simulink model "Project_Controller"  (R2025b)
settings: Solver=FixedStepDiscrete  StartTime=0.0  StopTime=36  FixedStep=1e-4  RelTol=1e-3
model workspace (MATLAB code in the model file):
  | %% Model workspace of Project_Controller.slx (Data source: MATLAB Code)
  | % The whole design chain, so the model runs on its own: physical parameters -> state-space model
  | % -> LQR with integral action -> Kalman filter -> discretization. Needs Control System Toolbox.
  | % Same computation as plant_model.m + controller_design.m (gain set v3a) + controller_params.m.
  | % build_controller_model.m copies this file into the model and checks it against those files.
  | 
  | %% Test case (same controller for both, no retuning)
  | rHigh = 0.015;   % [m] 0.015 (15 -> 5 mm) or 0.020 (20 -> 5 mm)
  | rLow  = 0.005;   % [m]
  | tHold = 12;      % [s] rLow, rHigh, rLow for tHold s each (stop time = 3*tHold = 36 s)
  | 
  | %% Physical parameters (project description, Table 1)
  | R    = 0.55;      % motor resistance [Ohm]
  | L    = 0.8e-3;    % motor inductance [H]
  | ki   = 0.036;     % torque constant [Nm/A]
  | kb   = 0.036;     % back-emf constant [V/(rad/s)]
  | lead = 0.01;      % ball screw lead [m/rev]
  | eta  = 1;         % ball screw efficiency (prescribed; real value < 1, robustness checked)
  | ma   = 0.3;       % actuator moving mass [kg]
  | ml   = 0.51;      % payload mass [kg]
  | 
  | %% Identified parameters (Section 3 of the report)
  | ks   = 131.66;    % spring [N/m], static stretch test
  | bs   = 0.0048;    % damper [Ns/m], free decay, logarithmic decrement
  | kv   = 0.99;      % input gain relative to Table 1, closed-loop frequency response
  | tauM = 0.018;     % actuator time constant [s], frequency response (Table 1 gives 31 ms)
  | tauS = 0.0106;    % sensor lag [s], Balluff -3 dB at 15 Hz
  | 
  | %% State-space model, deviations from the equilibrium point (plant_model.m)
  | % states [i y ydot x xdot xs]: current, actuator pos/vel, payload pos/vel, sensor state
  | N  = 2*pi/lead;             % screw ratio, omega = N*ydot [rad/m]
  | Kf = eta*N*ki;              % actuator force per ampere [N/A]
  | Kb = kb*N;                  % back emf per actuator speed [V/(m/s)]
  | Me = tauM*Kf*Kb/R;          % effective moving mass that gives tauM = Me*R/(Kf*Kb) [kg]
  | A = [ -R/L     0       -Kb/L     0       0        0
  |          0     0         1       0       0        0
  |      Kf/Me -ks/Me    -bs/Me   ks/Me   bs/Me       0
  |          0     0         0       0       1        0
  |          0  ks/ml     bs/ml  -ks/ml  -bs/ml       0
  |          0     0         0   1/tauS      0  -1/tauS ];
  | B = [kv/L; 0; 0; 0; 0; 0];
  | C = [0 0 0 0 0 1];          % only the (lagged) payload position is measured
  | n = size(A, 1);
  | 
  | %% LQR with integral action (L3d, L3g), Bryson's rule q_ii = 1/x_max^2, r = 1/u_max^2
  | % max: i 5 A, y 25 mm (stroke), ydot 0.15 m/s, x 8 mm, xdot 20 mm/s, xs not weighted,
  | % integral 1 mm*s, voltage 5 V
  | Ai = [A zeros(n, 1); -C 0];
  | Bi = [B; 0];
  | Q  = diag(1 ./ [5 0.025 0.15 0.008 0.02 1e3 0.001].^2);
  | Ru = 1/5^2;
  | Kaug = lqr(Ai, Bi, Q, Ru);
  | K  = Kaug(1:n);             % u = -K*xhat + Ke*xN
  | Ke = -Kaug(n + 1);
  | 
  | %% Kalman filter (LQE, L3h): process noise as voltage (3 V) and payload force (1 N push)
  | G   = [B, [0; 0; 0; 0; 1/ml; 0]];
  | sigX = 22e-6;               % measured sensor noise std [m]
  | [~, Lobs] = kalman(ss(A, [B G], C, 0), diag([3^2, 1^2]), sigX^2);
  | 
  | %% Discretization at the Speedgoat rate. Observer inputs [u; x]
  | Ts = 1e-4;                  % [s]
  | obsD = c2d(ss(A - Lobs*C, [B Lobs], eye(n), 0), Ts);
  | Ao = obsD.A;  Bo = obsD.B;
  | 
  | %% Holding voltage (equilibrium input) and voltage limit
  | vMax   = 5;                 % interface limit [V]
  | vBias  = 0.6;               % measured holding voltage [V]
  | uLim   = [-vMax, vMax];     % limit on u + vBias [V]
  | 
  | %% Reference prefilter 1/(tauPre*s + 1)^2, outside the loop
  | tauPre = 0.3;               % [s]
  | preD = ss(c2d(tf(1, [tauPre^2 2*tauPre 1]), Ts));
  | 
  | %% Start-up from the measured rest position x(0) (it changes between sessions, 1.57-1.85 mm)
  | x0map  = [0; 1; 0; 1; 0; 1];                     % xhat0 = x0map*x(0): positions = x(0), rest
  | preMap = (eye(size(preD.A)) - preD.A) \ preD.B;   % prefilter state in steady state at x(0)
  | 
  | %% Chirp excitation (frequency-response identification) and dither: both off
  | aExc = 0;  tExc = 5;  tExcDur = 60;  fExc1 = 0.3;  fExc2 = 20;
  | aDither = 0;  fDither = 100;
undefined symbols (not defined in the file): DiscIntNeverNeededParam, Pull, up
libraries: speedgoatlib_IO183 x3, simulink x1
settings Model: SimulationMode=external  Creator=rafaeltavares  LastModifiedBy=havard
settings SolverCC: ConcurrentTasks=on  AlgebraicLoopSolver=TrustRegion  PositivePriorityOrder=on  InsertRTBMode=Never (minimum delay)
settings DataIOCC: SaveFormat=StructureWithTime  ReturnWorkspaceOutputs=off
settings OptimizationCC: BlockReduction=off  OptimizeBlockIOStorage=off  BufferReuse=off  GlobalBufferReuse=off  ExpressionFolding=off  LocalBlockOutputs=off  OptimizeDataStoreBuffers=off  BusAssignmentInplaceUpdate=off
settings DebuggingCC: TasksWithSamePriorityMsg=none  UnconnectedInputMsg=warning  UnconnectedOutputMsg=warning  UnconnectedLineMsg=warning  UnderSpecifiedDimensionMsg=warning  ArithmeticOperatorsInVariantConditions=warning
settings HardwareCC: ProdBitPerLong=64.0  ProdLongLongMode=on  ProdHWDeviceType=Intel->x86-64 (Linux 64)
settings ModelReferenceCC: EnableRefExpFcnMdlSchedulingChecks=on
settings SFSimCC: CustomCodeUndefinedFunction=UseInterfaceOnly
settings RTWCC: SystemTargetFile=speedgoat.tlc  TemplateMakefile=slrealtime_default_tmf  Toolchain=Simulink Real-Time Toolchain  BuildConfiguration=Faster Runs  CodeExecutionProfiling=on  TargetLang=C++  GPUComputeCapability=3.5  DLArmComputeVersion=19.05  Description=Speedgoat Real-Time Target Machine
settings SimulinkRealTimeTargetCC: SLRTFileLogMaxRuns=1.0  ExtModeMaxTrigDuration=10.0  ExtModeStaticAllocSize=1000000.0  ExtModeTransport=0.0  MultiwordLength=2048.0  DynamicStringBufferSize=256.0  PreserveMATLABNamespacesInGeneratedCode=on  SubcomponentCodeInterfacePackaging=Reusable function  InstructionSetFMA=off  LogToMDFFile=off

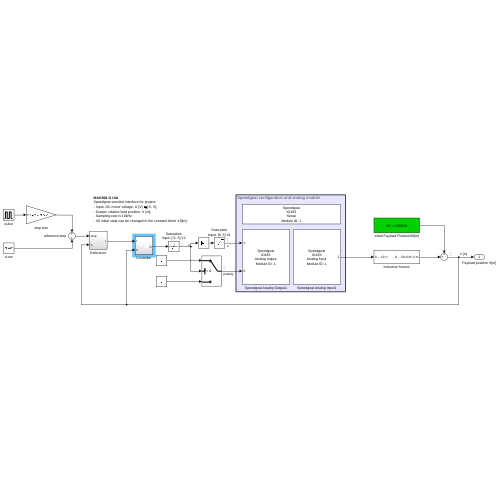
[thumbnail: Simulink's stored preview of the top-level diagram]
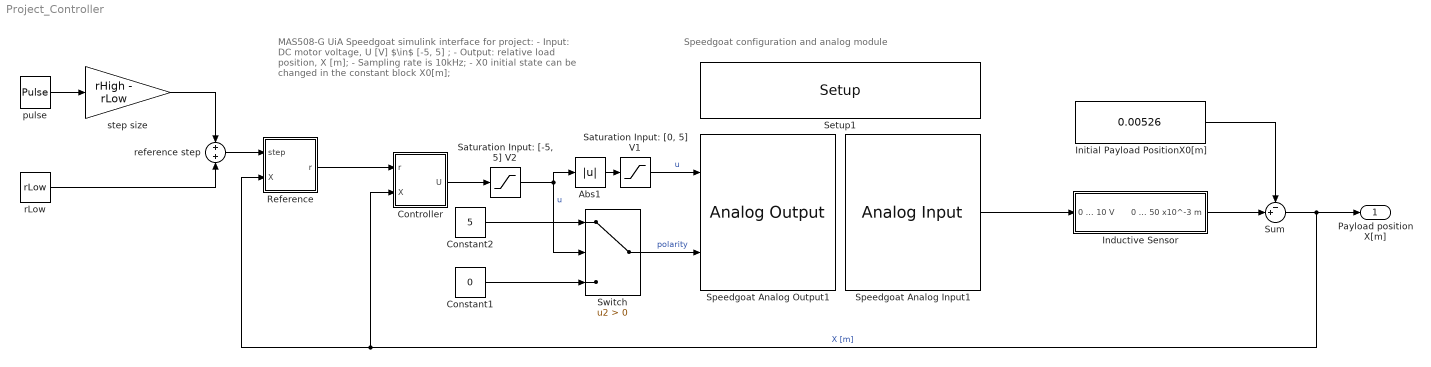
== system Project_Controller ==
  note: MAS508-G UiA
      | Speedgoat simulink interface for project:
      | - Input: DC motor voltage, U [V] $\in$ [-5, 5] ;
      | - Output: relative load position, X [m];
      | - Sampling rate is 10kHz;
      | - X0 initial state can be changed in the constant block X0[m];
  note: Speedgoat configuration and analog module
  Abs1 : Abs  SaturateOnIntegerOverflow=off
  Constant1 : Constant  Value=0
  Constant2 : Constant  Value=5
  Controller : Subsystem
  "Inductive Sensor " : Subsystem
  "Initial Payload PositionX0[m] " : Constant  Value=0.00526
      mask Display:
      | set_param(gcb,'BackgroundColor','green');
      | fprintf('X0 = %s', get_param(gcb,'Value'))
  Reference : Subsystem
  "Saturation Input: [-5, 5] V2" : Saturate  UpperLimit=5  LowerLimit=-5
  "Saturation Input: [0, 5] V1" : Saturate  UpperLimit=5  LowerLimit=0
  Setup1 : speedgoatlib_IO183/Setup  parModuleId=1  parPciSlot=-1  parDaSimult=on  parAdCoupling=Single Ended  parAdRange=0..10V  parAdChannelLow=1  parAdChannelHigh=1  parDaChannels=[1 2]  parDaRange=0..5V  parDaInit=[0 5 0 0]  parDaReset=1  parDoChannels=[1:8]  parDoInit=[0]  parDoReset=[1]  parDiChannels=[9:16]  parIOPullReferenceFront=Pull-up (3.3V)  parIOPullReferenceRear=Pull-up (3.3V)
      settings: SourceProductName=IO183
  Speedgoat Analog Input1 : speedgoatlib_IO183/Analog Input  Priority=0  parModuleId=1  parSampTime=-1  parPciSlot=-1  parAdChannelLow=1  parAdChannelHigh=1
      settings: SourceProductName=IO183
  Speedgoat Analog Output1 : speedgoatlib_IO183/Analog Output  parModuleId=1  parSampTime=-1  parDaSimult=on  parPciSlot=-1  parDaChannels=[1 2]  parDaInit=[0 5 0 0]  parDaReset=[1 1 1 1]
      settings: SourceProductName=IO183
  Sum : Sum  Inputs=-+|
  Switch : Switch  Criteria=u2 > Threshold  SaturateOnIntegerOverflow=off  InputSameDT=off
  pulse : DiscretePulseGenerator  PulseType=Time based  Period=2*tHold  PulseWidth=50  PhaseDelay=tHold
  rLow : Constant  Value=rLow
  reference step : Sum
  step size : Gain  Gain=rHigh - rLow
  Payload position X[m] : Outport
  wires:
  "Inductive Sensor "/1(0 ... 50 x10^-3 m) -> Sum/2
  "Initial Payload PositionX0[m] "/1 -> Sum/1
  "Saturation Input: [0, 5] V1"/1 -> Speedgoat Analog Output1/1  "u"
  Constant2/1 -> Switch/1
  Speedgoat Analog Input1/1 -> "Inductive Sensor "/1(0 ... 10 V)
  Abs1/1 -> "Saturation Input: [0, 5] V1"/1
  Switch/1 -> Speedgoat Analog Output1/2  "polarity"
  Constant1/1 -> Switch/3
  "Saturation Input: [-5, 5] V2"/1 -> Abs1/1, Switch/2  "u"
  Sum/1 -> Reference/2(X), Controller/2(X), Payload position X[m]/1  "X [m]"
  pulse/1 -> step size/1
  step size/1 -> reference step/1
  rLow/1 -> reference step/2
  reference step/1 -> Reference/1(step)
  Reference/1(r) -> Controller/1(r)
  Controller/1(U) -> "Saturation Input: [-5, 5] V2"/1

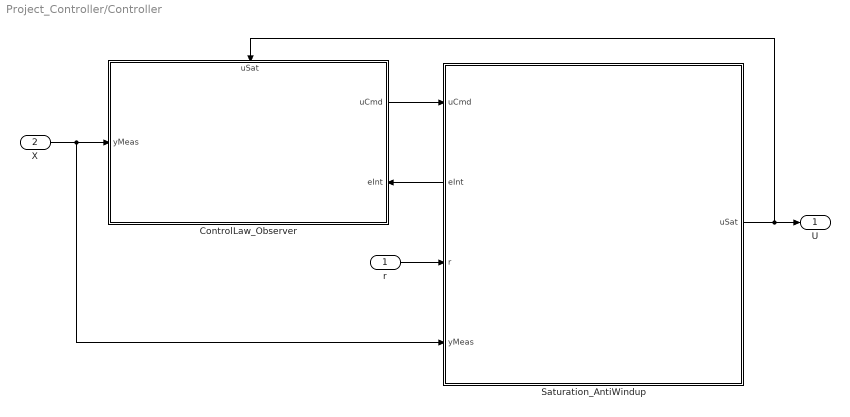
== system Project_Controller/Controller ==
  r : Inport
  X : Inport  Port=2
  ControlLaw_Observer : Subsystem
      settings: PortSchema="{\"entries\":[{\"content\":{\"sides\":[{\"content\":{\"connectorIds\":[\"In1\"]},\"type\":\"ConnectorPlacement.EquallySpacedRectSide\",\"uuid\":\"4ab0fcb8-52c7-4a4e-9377-be86be06758b\"},{\"content\":{\"connectorIds\":[\"Out1\",\"In3\"],\"side\":\"RIGHT\"},\"type\":\"ConnectorPlacement.EquallySpacedRectSide\",\"uuid\":\"0c93ed77-db89-4914-8ed3-cc59a8eb3b85\"},{\"content\":{\"connectorIds\":[\"In2\"],\"side\":\"TOP\"},\"type\":\"ConnectorPlacement.EquallySpacedRectSide\",\"uuid\":\"1c748175-366b-4d57-8d03-3856bbcdfb09\"},{\"content\":{\"side\":\"BOTTOM\"},\"type\":\"ConnectorPlacement.EquallySpacedRectSide\",\"uuid\":\"18ee6780-29bb-4133-baad-5bb614cd70f7\"}]},\"type\":\"ConnectorPlacement.EquallySpacedConnector\",\"uuid\":\"9b829baf-7a37-4ed0-ad0c-dec2a53cf1cf\"}],\"packageUris\":[\"http://schema.mathworks.com/mf0/Connector/R2020b\"],\"version\":\"1.0\"}"
  Saturation_AntiWindup : Subsystem
      settings: PortSchema="{\"entries\":[{\"content\":{\"sides\":[{\"content\":{\"connectorIds\":[\"In1\",\"Out2\",\"In2\",\"In3\"]},\"type\":\"ConnectorPlacement.EquallySpacedRectSide\",\"uuid\":\"fd51be67-1b16-4c80-8941-43d479349b34\"},{\"content\":{\"connectorIds\":[\"Out1\"],\"side\":\"RIGHT\"},\"type\":\"ConnectorPlacement.EquallySpacedRectSide\",\"uuid\":\"50a9a10a-2e08-446e-b14e-5678e3c6d1e3\"},{\"content\":{\"side\":\"TOP\"},\"type\":\"ConnectorPlacement.EquallySpacedRectSide\",\"uuid\":\"8fd36ea3-ab38-479f-a719-6e347c4892f4\"}]},\"type\":\"ConnectorPlacement.EquallySpacedConnector\",\"uuid\":\"95e37cf3-826c-49dc-833f-2565447af58e\"}],\"packageUris\":[\"http://schema.mathworks.com/mf0/Connector/R2020b\"],\"version\":\"1.0\"}"
  U : Outport
  wires:
  r/1 -> Saturation_AntiWindup/2(r)
  X/1 -> ControlLaw_Observer/1(yMeas), Saturation_AntiWindup/3(yMeas)
  ControlLaw_Observer/1(uCmd) -> Saturation_AntiWindup/1(uCmd)
  Saturation_AntiWindup/1(uSat) -> U/1, ControlLaw_Observer/2(uSat)
  Saturation_AntiWindup/2(eInt) -> ControlLaw_Observer/3(eInt)

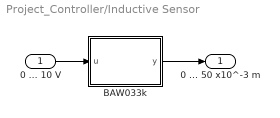
== system Project_Controller/Inductive Sensor  ==
  0 ... 10 V : Inport
  BAW033k : MATLAB Function  TreatAsAtomicUnit=on
  0 ... 50 x10^-3 m : Outport  VectorParamsAs1DForOutWhenUnconnected=off
  wires:
  BAW033k/1(y) -> 0 ... 50 x10^-3 m/1
  0 ... 10 V/1 -> BAW033k/1(u)

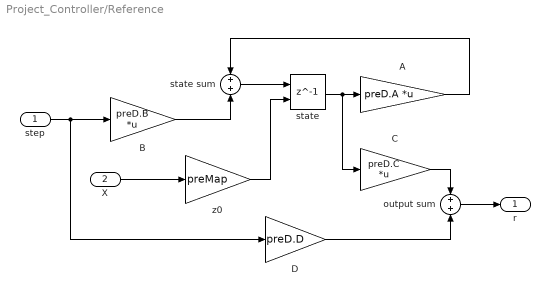
== system Project_Controller/Reference ==
  step : Inport
  X : Inport  Port=2
  A : Gain  Gain=preD.A  Multiplication=Matrix(K*u)
  B : Gain  Gain=preD.B  Multiplication=Matrix(K*u)
  C : Gain  Gain=preD.C  Multiplication=Matrix(K*u)
  D : Gain  Gain=preD.D
  output sum : Sum
  state : Delay  DelayLength=1  InitialConditionSource=Input port  SampleTime=Ts
      settings: InputPortMap=u0,p4
  state sum : Sum
  z0 : Gain  Gain=preMap
  r : Outport
  wires:
  output sum/1 -> r/1
  A/1 -> state sum/1
  state/1 -> C/1, A/1
  z0/1 -> state/2
  X/1 -> z0/1
  C/1 -> output sum/1
  D/1 -> output sum/2
  B/1 -> state sum/2
  state sum/1 -> state/1
  step/1 -> B/1, D/1

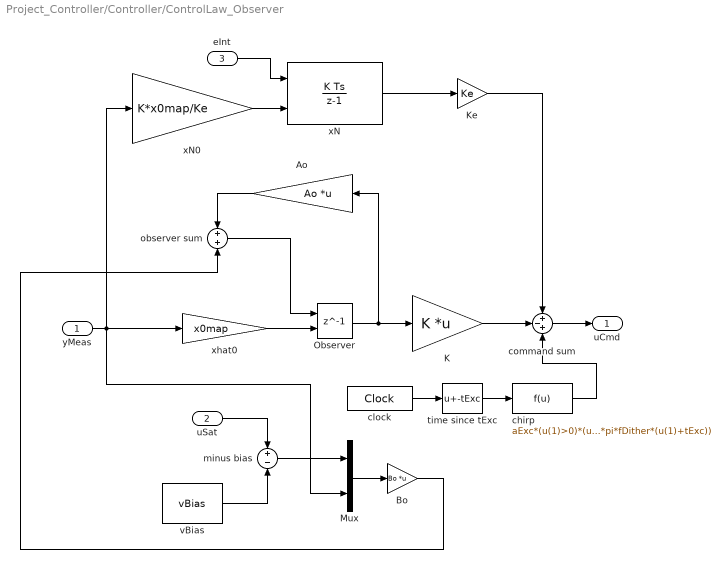
== system Project_Controller/Controller/ControlLaw_Observer ==
  yMeas : Inport
  uSat : Inport  Port=2
  eInt : Inport  Port=3
  Ao : Gain  Gain=Ao  Multiplication=Matrix(K*u)
  Bo : Gain  Gain=Bo  Multiplication=Matrix(K*u)
  K : Gain  Gain=K  Multiplication=Matrix(K*u)
  Ke : Gain  Gain=Ke
  Mux : Mux  Inputs=2
  Observer : Delay  DelayLength=1  InitialConditionSource=Input port  SampleTime=Ts
      settings: InputPortMap=u0,p4
  chirp : Fcn  Expr=aExc*(u(1)>0)*(u(1)<tExcDur)*sin(2*pi*(fExc1*u(1) + (fExc2-fExc1)/(2*tExcDur)*u(1)^2)) + aDither*sin(2*pi*fDither*(u(1)+tExc))
  clock : DigitalClock  SampleTime=Ts
  command sum : Sum  Inputs=+-+
  minus bias : Sum  Inputs=+-
  observer sum : Sum
  time since tExc : Bias  Bias=-tExc  SaturateOnIntegerOverflow=off
  vBias : Constant  Value=vBias
  xN : DiscreteIntegrator  InitialConditionSource=external  SampleTime=Ts  ICPrevOutput=DiscIntNeverNeededParam  ICPrevScaledInput=DiscIntNeverNeededParam
  xN0 : Gain  Gain=K*x0map/Ke
  xhat0 : Gain  Gain=x0map
  uCmd : Outport
  wires:
  Ke/1 -> command sum/1
  eInt/1 -> xN/1
  xhat0/1 -> Observer/2
  yMeas/1 -> Mux/2, xhat0/1, xN0/1
  command sum/1 -> uCmd/1
  Observer/1 -> Ao/1, K/1
  xN0/1 -> xN/2
  Ao/1 -> observer sum/1
  xN/1 -> Ke/1
  K/1 -> command sum/2
  observer sum/1 -> Observer/1
  uSat/1 -> minus bias/1
  vBias/1 -> minus bias/2
  minus bias/1 -> Mux/1
  Mux/1 -> Bo/1
  Bo/1 -> observer sum/2
  time since tExc/1 -> chirp/1
  chirp/1 -> command sum/3
  clock/1 -> time since tExc/1

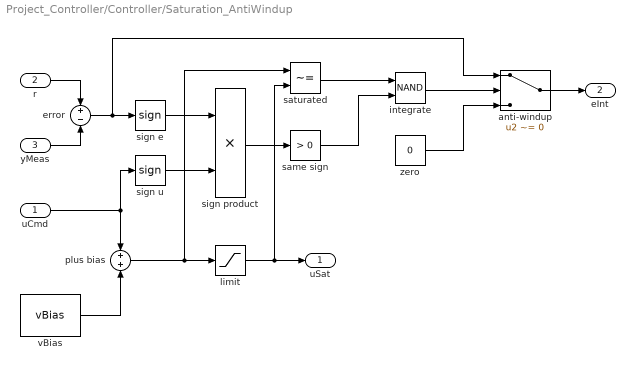
== system Project_Controller/Controller/Saturation_AntiWindup ==
  uCmd : Inport
  r : Inport  Port=2
  yMeas : Inport  Port=3
  anti-windup : Switch  Criteria=u2 ~= 0  SaturateOnIntegerOverflow=off  InputSameDT=off
  error : Sum  Inputs=+-
  integrate : Logic  Operator=NAND  AllPortsSameDT=off  OutDataTypeStr=boolean
  limit : Saturate  UpperLimit=uLim(2)  LowerLimit=uLim(1)
  plus bias : Sum
  same sign : simulink/Logic and Bit Operations/Compare To Constant  relop=>  const=0  OutDataTypeStr=boolean
  saturated : RelationalOperator  Operator=~=  OutDataTypeStr=boolean  RndMeth=Simplest  InputSameDT=off
  sign e : Signum
  sign product : Product
  sign u : Signum
  vBias : Constant  Value=vBias
  zero : Constant  Value=0
  uSat : Outport
  eInt : Outport  Port=2
  wires:
  same sign/1 -> integrate/2
  sign u/1 -> sign product/2
  integrate/1 -> anti-windup/2
  yMeas/1 -> error/2
  saturated/1 -> integrate/1
  anti-windup/1 -> eInt/1
  uCmd/1 -> plus bias/1, sign u/1
  sign product/1 -> same sign/1
  r/1 -> error/1
  plus bias/1 -> limit/1, saturated/1
  sign e/1 -> sign product/1
  error/1 -> anti-windup/1, sign e/1
  zero/1 -> anti-windup/3
  limit/1 -> saturated/2, uSat/1
  vBias/1 -> plus bias/2

== matlab function Project_Controller/Inductive Sensor /BAW033k ==
  data: u input; y output
function y = fcn(u)
% Input: 0 ... 10 V
% Output: 0 ... 40 mm
y =(40*10^-3/10)*u; %Output in SI [m]
